simulink model "Resonant_Load_PID"  (R2024b)
settings: Solver=ode5  StartTime=0.0  StopTime=1.5  FixedStep=1e-03  RelTol=1e-3
undefined symbols (not defined in the file): DiscIntNeverNeededParam, Kd, Ki, Kp, Kw, National_Instruments, PCI, sens, T_sim, TL
libraries: sldrtlib x3, simulink x1
settings Model: SimulationMode=external  ExtModeTrigDuration=45001  Creator=lenovo  LastModifiedBy=aboulenien
settings DataIOCC: ReturnWorkspaceOutputs=off
settings HardwareCC: ProdBitPerLong=64  ProdHWDeviceType=Intel->x86-64 (Linux 64)
settings RTWCC: Description=Simulink Desktop Real-Time  SystemTargetFile=sldrt.tlc  TemplateMakefile=sldrt.tmf  RTWCompilerOptimization=on
settings CodeAppCC: MaxIdLength=95
settings SimulinkDesktopRealTimeCC: TargetLibSuffix=_sldrt.a  TargetPreCompLibLocation=C:\Program Files\MATLAB\R2024b\toolbox\sldrt\lib\win64  ParMdlRefBuildCompliant=on

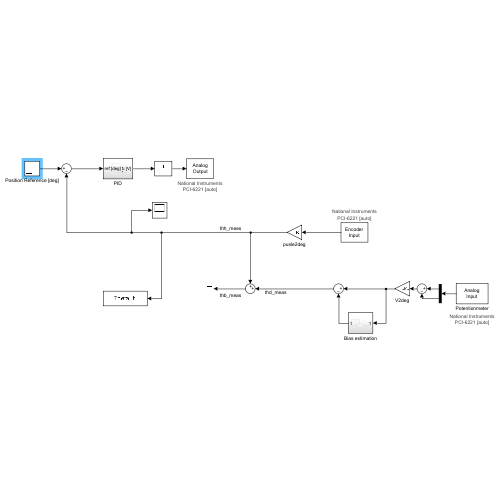
[thumbnail: Simulink's stored preview of the top-level diagram]
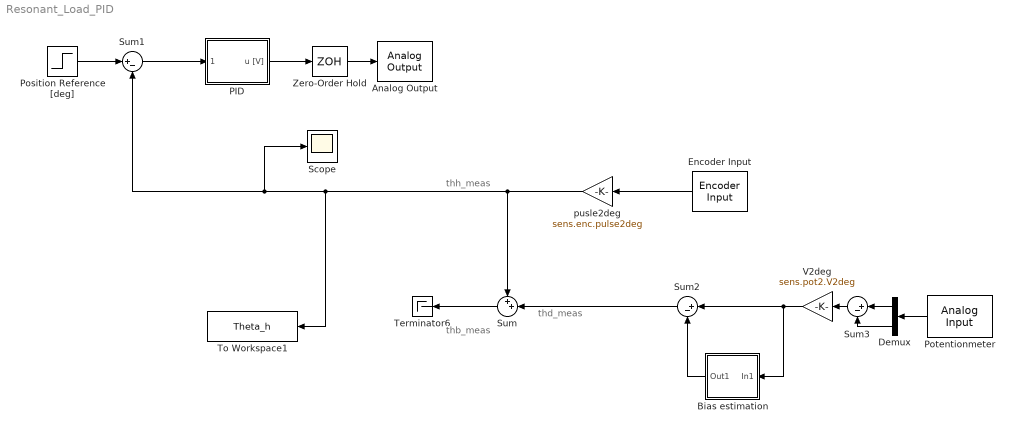
== system Resonant_Load_PID ==
  note: thh_meas
  note: thb_meas
  note: thd_meas
  Analog Output : sldrtlib/Analog Output  SampleTime=-1  MaxMissedTicks=10  ShowMissedTicks=off  YieldWhenWaiting=off  DrvName=National_Instruments/PCI-6221  DrvAddress=4294967295  DrvOptions=[0 0 0 2 0]  Channels=1  RangeMode=1  VoltRange=1  InitialValue=0  FinalValue=0
      settings: AttributesFormatString=National Instruments\nPCI-6221 [auto]
  Bias estimation : Subsystem
  Demux : Demux  Outputs=2
  Encoder Input : sldrtlib/Encoder Input  SampleTime=T_sim  MaxMissedTicks=10  ShowMissedTicks=off  YieldWhenWaiting=off  DrvName=National_Instruments/PCI-6221  DrvAddress=4294967295  DrvOptions=[0 0 0 2 0]  Channels=1  QuadMode=3  IndexPulse=1  InputFilter=Inf  DataType=1
      settings: AttributesFormatString=National Instruments\nPCI-6221 [auto]
  PID : Subsystem
  Position Reference [deg] : Step  After=120  SampleTime=0
  Potentionmeter : sldrtlib/Analog Input  SampleTime=0.1  MaxMissedTicks=10  ShowMissedTicks=off  YieldWhenWaiting=off  DrvName=National_Instruments/PCI-6221  DrvAddress=4294967295  DrvOptions=[0 0 0 2 0]  Channels=[3 4]  RangeMode=1  VoltRange=2  DataType=1
      settings: AttributesFormatString=National Instruments\nPCI-6221 [auto]
  Scope : Scope
  Sum : Sum  Inputs=++|
  Sum1 : Sum  Inputs=|+-
  Sum2 : Sum  Inputs=|+-
  Sum3 : Sum  Inputs=|+-
  Terminator6 : Terminator
  To Workspace1 : ToWorkspace  VariableName=Theta_h  SaveFormat=Structure With Time  SampleTime=0.001
  V2deg : Gain  Gain=sens.pot2.V2deg
  Zero-Order Hold : ZeroOrderHold  SampleTime=T_sim
  pusle2deg : Gain  Gain=sens.enc.pulse2deg
  wires:
  Zero-Order Hold/1 -> Analog Output/1
  Sum2/1 -> Sum/2
  Sum1/1 -> PID/1(ref [deg])
  pusle2deg/1 -> To Workspace1/1, Scope/1, Sum1/2, Sum/1
  Sum/1 -> Terminator6/1
  Position Reference [deg]/1 -> Sum1/1
  PID/1(u [V]) -> Zero-Order Hold/1
  Encoder Input/1 -> pusle2deg/1
  Bias estimation/1(Out1) -> Sum2/2
  Potentionmeter/1 -> Demux/1
  Demux/1 -> Sum3/1
  Demux/2 -> Sum3/2
  Sum3/1 -> V2deg/1
  V2deg/1 -> Bias estimation/1(In1), Sum2/1

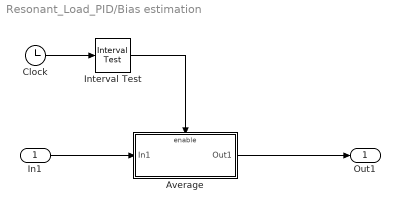
== system Resonant_Load_PID/Bias estimation ==
  In1 : Inport
  Average : Subsystem  TreatAsAtomicUnit=on
  Clock : Clock
  Interval Test : simulink/Logic and Bit Operations/Interval Test  IntervalClosedRight=on  uplimit=0.7  IntervalClosedLeft=on  lowlimit=0.2  OutDataTypeStr=boolean
  Out1 : Outport
  wires:
  In1/1 -> Average/1(In1)
  Average/1(Out1) -> Out1/1
  Clock/1 -> Interval Test/1
  Interval Test/1 -> Average/Enable

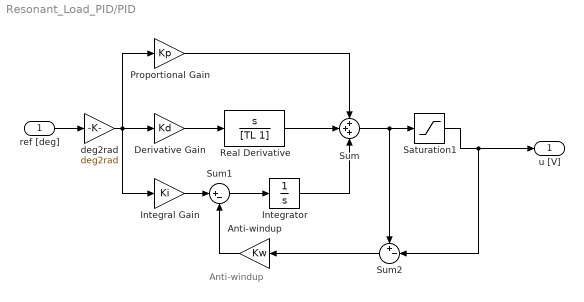
== system Resonant_Load_PID/PID ==
  note: Anti-windup
  ref [deg] : Inport
  Anti-windup : Gain  Gain=Kw
  Derivative Gain : Gain  Gain=Kd
  Integral Gain : Gain  Gain=Ki
  Integrator : Integrator
  Proportional Gain : Gain  Gain=Kp
  Real Derivative : TransferFcn  Numerator=[1 0]  Denominator=[TL 1]
  Saturation1 : Saturate  UpperLimit=12  LowerLimit=-12
  Sum : Sum  Inputs=+++
  Sum1 : Sum  Inputs=|+-
  Sum2 : Sum  Inputs=+-|
  deg2rad : Gain  Gain=deg2rad
  u [V] : Outport
  wires:
  Integrator/1 -> Sum/3
  Real Derivative/1 -> Sum/2
  Derivative Gain/1 -> Real Derivative/1
  Proportional Gain/1 -> Sum/1
  ref [deg]/1 -> deg2rad/1
  deg2rad/1 -> Proportional Gain/1, Integral Gain/1, Derivative Gain/1
  Sum/1 -> Saturation1/1, Sum2/1
  Saturation1/1 -> Sum2/2, u [V]/1
  Integral Gain/1 -> Sum1/1
  Anti-windup/1 -> Sum1/2
  Sum2/1 -> Anti-windup/1
  Sum1/1 -> Integrator/1

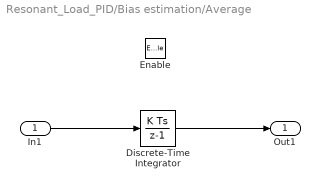
== system Resonant_Load_PID/Bias estimation/Average ==
  In1 : Inport
  Enable : EnablePort
  Discrete-Time Integrator : DiscreteIntegrator  gainval=2  SampleTime=-1  ICPrevOutput=DiscIntNeverNeededParam  ICPrevScaledInput=DiscIntNeverNeededParam
  Out1 : Outport
  wires:
  In1/1 -> Discrete-Time Integrator/1
  Discrete-Time Integrator/1 -> Out1/1
